simulink model "CHB_Rectifier"  (R2023b)
settings: Solver=FixedStepAuto  StartTime=0.0  StopTime=0.5  RelTol=1e-3
libraries: spsSeriesRLCBranchLib x4, spsVoltageMeasurementLib x4, spsMeanLib x3, spsParallelRLCBranchLib x2, spsUniversalBridgeLib x2, spsACVoltageSourceLib x1, spsCurrentMeasurementLib x1, slpidlib x1, powerlib_extras x1, spsRMSLib x1, spsTHDLib x1, spspowerguiLib x1
settings Model: SimulationMode=accelerator  Creator=abc6820292  LastModifiedBy=Epiphanye
settings SolverCC: ZeroCrossControl=EnableAll  ZeroCrossAlgorithm=Adaptive
settings DataIOCC: ReturnWorkspaceOutputs=off  Refine=10
settings DebuggingCC: IgnoredZcDiagnostic=none  UnconnectedInputMsg=warning  UnconnectedOutputMsg=warning  UnconnectedLineMsg=warning
settings ModelReferenceCC: EnableRefExpFcnMdlSchedulingChecks=on
settings RTWCC: DLArmComputeVersion=19.05

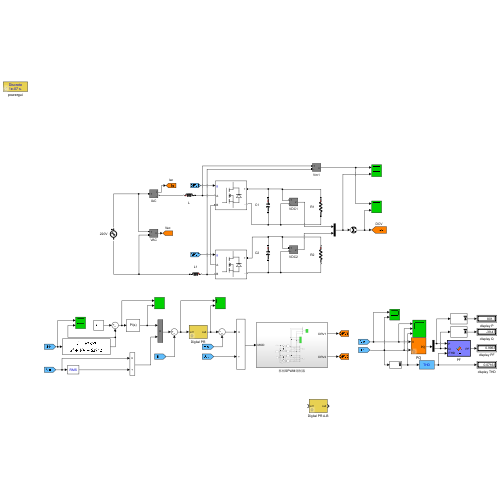
[thumbnail: Simulink's stored preview of the top-level diagram]
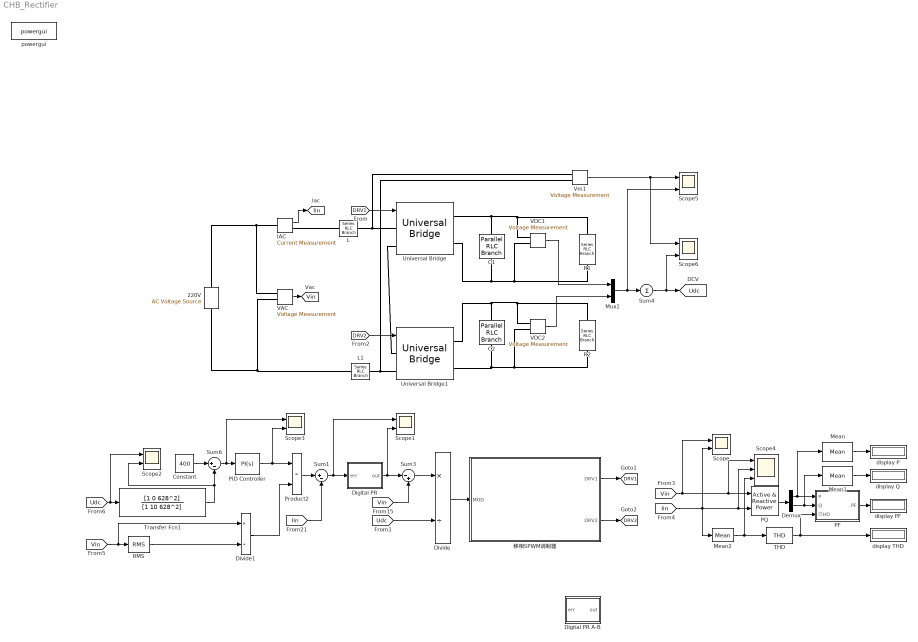
== system CHB_Rectifier ==
  220V : spsACVoltageSourceLib/AC Voltage Source  Amplitude=220*1.414  Phase=0  Frequency=50  SampleTime=0  Measurements=None  BusType=swing  Pref=10e3  Qref=0  Qmin=-inf  Qmax=+inf
  C1 : spsParallelRLCBranchLib/Parallel RLC Branch  LConnTagsString=a  RConnTagsString=__new0  BranchType=C  Resistance=1e3  Inductance=1e-3  SetiL0=off  InitialCurrent=0  Capacitance=1e-3  Setx0=on  InitialVoltage=80  Measurements=None
  C2 : spsParallelRLCBranchLib/Parallel RLC Branch  LConnTagsString=a  RConnTagsString=__new0  BranchType=C  Resistance=1e3  Inductance=1e-3  SetiL0=off  InitialCurrent=0  Capacitance=1e-3  Setx0=on  InitialVoltage=80  Measurements=None
  Constant : Constant  Value=400
  Demux : Demux  Outputs=2
  Digital PR : Subsystem  mask{Kp=8, Kr=100, Wc=5, Ts=1/40000, Upper=400, Lower=-400}
      mask DialogControl ParameterGroupVar Prompt: 参数
  Digital PR A-B : Subsystem  mask{Kp=6, Kr=400, Wc=5, Ts=1/20000, Upper=500, Lower=-500}
      mask DialogControl ParameterGroupVar Prompt: 参数
  Divide : Product  Inputs=*/
  Divide1 : Product  Inputs=*/
  IAC : spsCurrentMeasurementLib/Current Measurement  PhasorSimulation=off  OutputType=Complex  PSBequivalent=0
  L : spsSeriesRLCBranchLib/Series RLC Branch  LConnTagsString=__new0  RConnTagsString=__new0  BranchType=L  Resistance=25  Inductance=4e-4  SetiL0=off  InitialCurrent=0  Capacitance=2e-3  Setx0=on  InitialVoltage=350  Measurements=None
  L1 : spsSeriesRLCBranchLib/Series RLC Branch  LConnTagsString=__new0  RConnTagsString=__new0  BranchType=L  Resistance=25  Inductance=4e-4  SetiL0=off  InitialCurrent=0  Capacitance=2e-3  Setx0=on  InitialVoltage=350  Measurements=None
  Mean : spsMeanLib/Mean  Freq=50  Vinit=0  Ts=0
  Mean1 : spsMeanLib/Mean  Freq=50  Vinit=0  Ts=0
  Mean2 : spsMeanLib/Mean  Freq=20000  Vinit=0  Ts=0
  Mux1 : Mux  Inputs=2
  PF : MATLAB Function  TreatAsAtomicUnit=on
  PID Controller : slpidlib/PID Controller  Controller=PI  Form=Parallel  TimeDomain=Continuous-time  UseExternalTs=off  SampleTime=-1  IntegratorMethod=Forward Euler  FilterMethod=Forward Euler  ControllerParametersSource=internal  P=0.1  I=50  UseKiTs=off  D=0.005  N=100  UseFilter=on  TunerSelectOption=Transfer Function Based (PID Tuner App)  InitialConditionSource=internal  InitialConditionForIntegrator=0  InitialConditionForFilter=0  DifferentiatorICPrevScaledInput=0  ExternalReset=none  TrackingMode=off  Kt=1  LimitOutput=off  SatLimitsSource=internal  UpperSaturationLimit=40  LowerSaturationLimit=-20  LinearizeAsGain=on  AntiWindupMode=clamping  Kb=1  LimitIntegrator=off  UpperIntegratorSaturationLimit=inf  LowerIntegratorSaturationLimit=-inf  POutMin=[]  POutMax=[]  IOutMin=[]  IOutMax=[]  DOutMin=[]  DOutMax=[]  NOutMin=[]  NOutMax=[]  SumOutMin=[]  SumOutMax=[]  SaturationOutMin=[]  SaturationOutMax=[]  PParamMin=[]  PParamMax=[]  IParamMin=[]  IParamMax=[]  DParamMin=[]  DParamMax=[]  NParamMin=[]  NParamMax=[]  KbParamMin=[]  KbParamMax=[]  KtParamMin=[]  KtParamMax=[]  KbOutMin=[]  KbOutMax=[]  KtOutMin=[]  KtOutMax=[]  IntegratorOutMin=[]  IntegratorOutMax=[]  FilterOutMin=[]  FilterOutMax=[]  SumI1OutMin=[]  SumI1OutMax=[]  SumI2OutMin=[]  SumI2OutMax=[]  SumI3OutMin=[]  SumI3OutMax=[]  SumI4OutMin=[]  SumI4OutMax=[]  SumDOutMin=[]  SumDOutMax=[]  DifferentiatorOutMin=[]  DifferentiatorOutMax=[]  FilterDiffOutCoefMin=[]  FilterDiffOutCoefMax=[]  ReciprocalOutMin=[]  ReciprocalOutMax=[]  SumDenOutMin=[]  SumDenOutMax=[]  SumNumOutMin=[]  SumNumOutMax=[]  DivideOutMin=[]  DivideOutMax=[]  UdiffTsProdOutMin=[]  UdiffTsProdOutMax=[]  NTsProdOutMin=[]  NTsProdOutMax=[]  UintegralTsProdOutMin=[]  UintegralTsProdOutMax=[]  UngainTsProdOutMin=[]  UngainTsProdOutMax=[]  ClampingZeroOutDataTypeStr=Inherit: Inherit via back propagation  ClampingZeroOutMin=[]  ClampingZeroOutMax=[]  FilterDenConstantOutDataTypeStr=Inherit: Inherit via back propagation  FilterDenConstantOutMin=[]  FilterDenConstantOutMax=[]  PCopyOutDataTypeStr=Inherit: Inherit via back propagation  PCopyOutMin=[]  PCopyOutMax=[]  NCopyOutDataTypeStr=Inherit: Inherit via back propagation  NCopyOutMin=[]  NCopyOutMax=[]  IntegratorContinuousStateAttributes=''  IntegratorStateMustResolveToSignalObject=off  IntegratorRTWStateStorageClass=Auto  FilterContinuousStateAttributes=''  FilterStateMustResolveToSignalObject=off  FilterRTWStateStorageClass=Auto  ParallelPVariant=InternalParameters  IdealPVariant=Disabled  IVariant=InternalParameters  DVariant=Disabled  IntegratorVariant=Continuous  SatVariant=Disabled  AWVariant=Passthrough  PCopyVariant=Disabled  TRVariant=Disabled  FdbkBlocksVariant=Forward  IdealPFdbkVariant=Disabled  SatFdbkVariant=Disabled  DerivativeFilterVariant=Disabled  NVariant=Disabled  NCopyVariant=Disabled_SignalSpec  FilterICVariant=Disabled  IntegratorICVariant=InternalICs  ExternalResetVariant=Disabled  TRSumVariant=Passthrough  SumFdbkVariant=Disabled  SumVariant=Sum_PI  TsampFilterVariant=InternalTs  TsampNgainVariant=Passthrough  TsampIntegralVariant=Disabled_SignalSpec  ExternalSaturationOutDataTypeStr=Inherit: Same as second input
  PQ : powerlib_extras/Measurements/Active & Reactive Power  f1=50
  Product2 : Product  RndMeth=Zero
  R1 : spsSeriesRLCBranchLib/Series RLC Branch  LConnTagsString=__new0  RConnTagsString=__new0  BranchType=R  Resistance=100  Inductance=0.1  SetiL0=off  InitialCurrent=0  Capacitance=2e-3  Setx0=on  InitialVoltage=350  Measurements=None
  R2 : spsSeriesRLCBranchLib/Series RLC Branch  LConnTagsString=__new0  RConnTagsString=__new0  BranchType=R  Resistance=100  Inductance=0.1  SetiL0=off  InitialCurrent=0  Capacitance=2e-3  Setx0=on  InitialVoltage=350  Measurements=None
  RMS : spsRMSLib/RMS  TrueRMS=on  Freq=60  RMSInit=120  Ts=0
  Scope{,1..3,5..6} (6 alike) : Scope  NumInputPorts=2
  Scope4 : Scope  NumInputPorts=3
  Sum1 : Sum  Inputs=|+-
  Sum3 : Sum  Inputs=|-+
  Sum4 : Sum  Inputs=+
  Sum6 : Sum  Inputs=|+-
  THD : spsTHDLib/THD  Freq=50  Ts=0
  Transfer Fcn1 : TransferFcn  Numerator=[1 0 628^2]  Denominator=[1 10 628^2]
  Universal Bridge : spsUniversalBridgeLib/Universal Bridge  Arms=2  SnubberResistance=1e5  SnubberCapacitance=inf  Device=MOSFET / Diodes  Ron=1e-3  Lon=0  ForwardVoltages="[  0  0  ]"  ForwardVoltage=0  GTOparameters=[ 10e-6 , 20e-6 ]  IGBTparameters=[ 1e-6 , 2e-6 ]  Measurements=None  Measurements_2=None  converterType=Rectifier
  Universal Bridge1 : spsUniversalBridgeLib/Universal Bridge  Arms=2  SnubberResistance=1e5  SnubberCapacitance=inf  Device=MOSFET / Diodes  Ron=1e-3  Lon=0  ForwardVoltages="[  0  0  ]"  ForwardVoltage=0  GTOparameters=[ 10e-6 , 20e-6 ]  IGBTparameters=[ 1e-6 , 2e-6 ]  Measurements=None  Measurements_2=None  converterType=Rectifier
  VAC : spsVoltageMeasurementLib/Voltage Measurement  PhasorSimulation=off  OutputType=Complex  PSBequivalent=0
  VDC1 : spsVoltageMeasurementLib/Voltage Measurement  PhasorSimulation=off  OutputType=Complex  PSBequivalent=0
  VDC2 : spsVoltageMeasurementLib/Voltage Measurement  PhasorSimulation=off  OutputType=Complex  PSBequivalent=0
  Vm1 : spsVoltageMeasurementLib/Voltage Measurement  PhasorSimulation=off  OutputType=Complex  PSBequivalent=0
  display P : Display
  display PF : Display
  display Q : Display
  display THD : Display
  powergui : spspowerguiLib/powergui  SimulationMode=Discrete  SampleTime=1e-7  frequency=60  Iterations=50  frequencyindice=0  Pbase=100e6  ErrMax=1e-4  UnitsV=kV  UnitsW=MW  buscounter=0  FunctionMessages=off  echomessages=off  EnableUseOfTLC=off  CurrentSourceSwitches=off  DisableSnubberDevices=off  DisableRonSwitches=off  DisableVfSwitches=off  DisplayEquations=off  AutomaticDiscreteSolvers=off  SolverType=Tustin/Backward Euler (TBE)  Interpol=off  ExternalGateDelay=off  methode=off  Ts=0  x0status=blocks  SPID=off  SwTol=0  HookPort=off  NonlinearTolerance=1e-4  nMaxIteration=100  ContinueOnMaxIteration=off  RestoreLinks=warning  ResistiveCurrentMeasurement=off  Frange=[0:2:500]  Ylog=off  Xlog=on  ShowGrid=off  save=off  variable=ZData  structure=QQQQQ  ZoomFFT=off  StartTime=0.5  cycles=15  DisplayStyle=1  fundamental=50  FreqAxis=off  MaxFrequency=1000  frequencyindicesteady=1  RmsSteady=1  display=off
  移相SPWM调制器 : Subsystem
  tag scope: DRV1=global, DRV2=global, Iin=global, Udc=global, Vin=global
  wires:
  VAC/1 -> [Vin]
  [Vin] -> Scope/1, Scope4/1, PQ/1
  PQ/1 -> Demux/1
  Demux/1 -> Mean/1, PF/1(P)
  Demux/2 -> Mean1/1, PF/2(Q)
  THD/1 -> display THD/1, PF/3(iTHD)
  PF/1(PF) -> display PF/1
  Mean/1 -> display P/1
  Mean1/1 -> display Q/1
  [DRV1] -> Universal Bridge/1
  移相SPWM调制器/1(DRV1) -> [DRV1]
  IAC/1 -> [Iin]
  [Iin] -> Scope/2, Mean2/1, Scope4/2, PQ/2
  Mean2/1 -> Scope4/3, THD/1
  Sum1/1 -> Digital PR/1(err), Scope1/1
  Product2/1 -> Sum1/1
  PID Controller/1 -> Scope3/2, Product2/1
  Sum3/1 -> Divide/1
  Sum6/1 -> Scope3/1, PID Controller/1
  Constant/1 -> Sum6/1
  Vm1/1 -> Scope6/1, Scope5/1
  [DRV2] -> Universal Bridge1/1
  VDC1/1 -> Mux1/1
  VDC2/1 -> Mux1/2
  Mux1/1 -> Scope5/2, Sum4/1
  Sum4/1 -> Scope6/2, [Udc]
  Digital PR/1(out) -> Scope1/2, Sum3/1
  [Udc] -> Divide/2
  移相SPWM调制器/2(DRV2) -> [DRV2]
  Divide/1 -> 移相SPWM调制器/1(MOD)
  [Vin] -> Sum3/2
  [Vin] -> Divide1/1, RMS/1
  RMS/1 -> Divide1/2
  Divide1/1 -> Product2/2
  [Iin] -> Sum1/2
  [Udc] -> Scope2/1, Transfer Fcn1/1
  Transfer Fcn1/1 -> Scope2/2, Sum6/2
  connections:
  Universal Bridge/RConn2 -- VDC1/LConn2 -- R1/RConn1 -- C1/RConn1
  IAC/LConn1 -- VAC/LConn1 -- 220V/RConn1
  C1/LConn1 -- R1/LConn1 -- VDC1/LConn1 -- Universal Bridge/RConn1
  L/RConn1 -- Universal Bridge/LConn1 -- Vm1/LConn1
  L/LConn1 -- IAC/RConn1
  L1/RConn1 -- 220V/LConn1 -- VAC/LConn2
  Universal Bridge/LConn2 -- Universal Bridge1/LConn1
  VDC2/LConn2 -- R2/RConn1 -- Universal Bridge1/RConn2 -- C2/RConn1
  C2/LConn1 -- Universal Bridge1/RConn1 -- VDC2/LConn1 -- R2/LConn1
  Vm1/LConn2 -- L1/LConn1 -- Universal Bridge1/LConn2

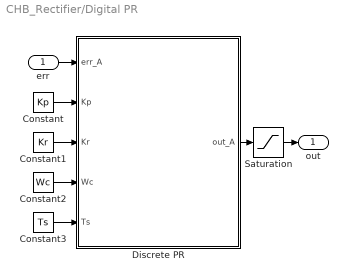
== system CHB_Rectifier/Digital PR ==
  err : Inport
  Constant : Constant  Value=Kp
  Constant1 : Constant  Value=Kr
  Constant2 : Constant  Value=Wc
  Constant3 : Constant  Value=Ts
  Discrete PR : MATLAB Function  TreatAsAtomicUnit=on
  Saturation : Saturate  UpperLimit=Upper  LowerLimit=Lower
  out : Outport
  wires:
  Constant1/1 -> Discrete PR/3(Kr)
  Constant3/1 -> Discrete PR/5(Ts)
  Constant/1 -> Discrete PR/2(Kp)
  Constant2/1 -> Discrete PR/4(Wc)
  Discrete PR/1(out_A) -> Saturation/1
  Saturation/1 -> out/1
  err/1 -> Discrete PR/1(err_A)

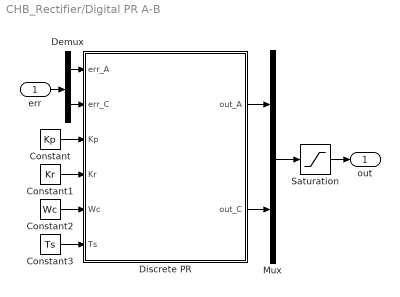
== system CHB_Rectifier/Digital PR A-B ==
  err : Inport
  Constant : Constant  Value=Kp
  Constant1 : Constant  Value=Kr
  Constant2 : Constant  Value=Wc
  Constant3 : Constant  Value=Ts
  Demux : Demux  Outputs=2
  Discrete PR : MATLAB Function  TreatAsAtomicUnit=on
  Mux : Mux  Inputs=2
  Saturation : Saturate  UpperLimit=Upper  LowerLimit=Lower
  out : Outport
  wires:
  Constant1/1 -> Discrete PR/4(Kr)
  Constant3/1 -> Discrete PR/6(Ts)
  Constant/1 -> Discrete PR/3(Kp)
  Constant2/1 -> Discrete PR/5(Wc)
  Demux/1 -> Discrete PR/1(err_A)
  err/1 -> Demux/1
  Demux/2 -> Discrete PR/2(err_C)
  Discrete PR/1(out_A) -> Mux/1
  Discrete PR/2(out_C) -> Mux/2
  Mux/1 -> Saturation/1
  Saturation/1 -> out/1

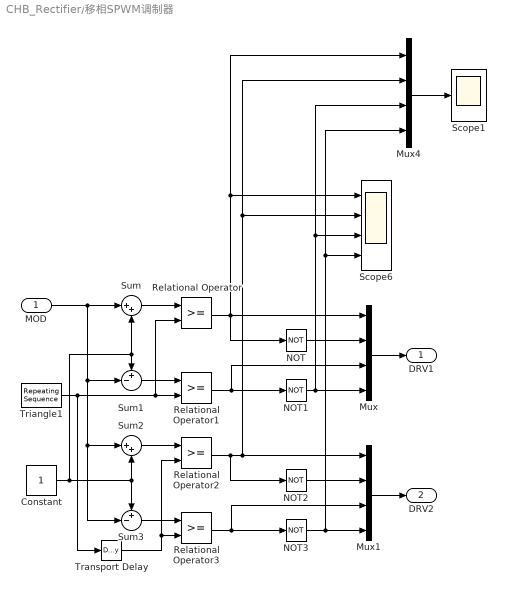
== system CHB_Rectifier/移相SPWM调制器 ==
  MOD : Inport
  Constant : Constant
  Mux : Mux
  Mux1 : Mux
  Mux4 : Mux
  NOT{,1..3} (4 alike) : Logic  Operator=NOT  IconShape=distinctive  AllPortsSameDT=off  OutDataTypeStr=boolean
  Relational Operator{,1..3} (4 alike) : RelationalOperator  OutDataTypeStr=boolean  InputSameDT=off
  Scope1 : Scope
  Scope6 : Scope  NumInputPorts=4
  Sum : Sum  Inputs=|++
  Sum1 : Sum  Inputs=+-|
  Sum2 : Sum  Inputs=|++
  Sum3 : Sum  Inputs=+-|
  Transport Delay : TransportDelay  DelayTime=1/20000/4
  Triangle1 : simulink/Sources/Repeating Sequence  rep_seq_t=[0 1/20000/2 1/20000]  rep_seq_y=[0 2 0]
  DRV1 : Outport
  DRV2 : Outport  Port=2
  wires:
  Triangle1/1 -> Transport Delay/1, Relational Operator1/2, Relational Operator/2
  Mux/1 -> DRV1/1
  NOT/1 -> Mux/2
  Relational Operator/1 -> Mux4/1, Scope6/1, Mux/1, NOT/1
  MOD/1 -> Sum3/2, Sum2/1, Sum1/2, Sum/1
  Sum/1 -> Relational Operator/1
  Sum1/1 -> Relational Operator1/1
  Relational Operator1/1 -> Mux/3, NOT1/1
  Constant/1 -> Sum3/1, Sum2/2, Sum/2, Sum1/1
  NOT1/1 -> Mux4/3, Scope6/3, Mux/4
  Relational Operator3/1 -> Mux1/3, NOT3/1
  Relational Operator2/1 -> Mux1/1, Mux4/2, Scope6/2, NOT2/1
  NOT2/1 -> Mux1/2
  NOT3/1 -> Mux4/4, Scope6/4, Mux1/4
  Sum3/1 -> Relational Operator3/1
  Sum2/1 -> Relational Operator2/1
  Transport Delay/1 -> Relational Operator3/2, Relational Operator2/2
  Mux1/1 -> DRV2/1
  Mux4/1 -> Scope1/1

== matlab function CHB_Rectifier/Digital PR/Discrete PR ==
  settings: updateMethod=DISCRETE  sampleTime=Ts
  data: err_A input; out_A output; Kp input; Kr input; Wc input; Ts input
function out_A  = fcn(err_A, Kp, Kr, Wc, Ts)

W0 = 50*2*pi;


persistent err_A1;
persistent err_A2;
persistent out_A1;
persistent out_A2;


%%对三相静态变量初始化
if isempty(err_A1)
    err_A1 = 0;
end
if isempty(err_A2)
    err_A2 = 0;
end
if isempty(out_A1)
    out_A1 = 0;
end
if isempty(out_A2)
    out_A2 = 0;
end


%%Discrete
t1 = Wc * Ts;
t2 = W0^2 * Ts^2;
t3 = t2 + 4*t1 + 4;

b0 = (Kp*t2 + 4*(Kp+Kr)*t1 + 4*Kp) / t3;
b1 = (2*Kp*t2 - 8*Kp) / t3;
b2 = (Kp*t2 + 4*Kp - 4*(Kp+Kr)*t1) / t3;
a1 = (2*t2 - 8) / t3;
a2 = (t2 - 4*t1 + 4) / t3;
%%限制输出
if b0>3000
    b0=0;
end
if b0<-3000
    b0=0;
end

%%计算输出量
out_A = b0*err_A + b1*err_A1 + b2*err_A2 - a1*out_A1 - a2*out_A2;
out_A2 = out_A1;
out_A1 = out_A;
err_A2 = err_A1;
err_A1 = err_A;

== matlab function CHB_Rectifier/PF ==
  data: P input; PF output; Q input; iTHD input
function PF = fcn(P,Q,iTHD)
% This block supports an embeddable subset of the MATLAB language.
% See the help menu for details. 
PF=(P/sqrt(P*P+Q*Q))/(sqrt(1+iTHD*iTHD));

== matlab function CHB_Rectifier/Digital PR A-B/Discrete PR ==
  settings: updateMethod=DISCRETE  sampleTime=Ts
  data: err_A input; err_C input; out_A output; Kp input; Kr input; Wc input; Ts input; out_C output
function [out_A, out_C] = fcn(err_A, err_C, Kp, Kr, Wc, Ts)

W0 = 50*2*pi;

%%定义三相静态变量
persistent err_A1;
persistent err_A2;
persistent out_A1;
persistent out_A2;

persistent err_C1;
persistent err_C2;
persistent out_C1;
persistent out_C2;

%%对三相静态变量初始化
if isempty(err_A1)
    err_A1 = 0;
end
if isempty(err_A2)
    err_A2 = 0;
end
if isempty(out_A1)
    out_A1 = 0;
end
if isempty(out_A2)
    out_A2 = 0;
end


if isempty(err_C1)
    err_C1 = 0;
end
if isempty(err_C2)
    err_C2 = 0;
end
if isempty(out_C1)
    out_C1 = 0;
end
if isempty(out_C2)
    out_C2 = 0;
end

%%Discrete
t1 = Wc * Ts;
t2 = W0^2 * Ts^2;
t3 = t2 + 4*t1 + 4;

b0 = (Kp*t2 + 4*(Kp+Kr)*t1 + 4*Kp) / t3;
b1 = (2*Kp*t2 - 8*Kp) / t3;
b2 = (Kp*t2 + 4*Kp - 4*(Kp+Kr)*t1) / t3;
a1 = (2*t2 - 8) / t3;
a2 = (t2 - 4*t1 + 4) / t3;

%%计算三相输出量
out_A = b0*err_A + b1*err_A1 + b2*err_A2 - a1*out_A1 - a2*out_A2;
out_A2 = out_A1;
out_A1 = out_A;
err_A2 = err_A1;
err_A1 = err_A;


out_C = b0*err_C + b1*err_C1 + b2*err_C2 - a1*out_C1 - a2*out_C2;
out_C2 = out_C1;
out_C1 = out_C;
err_C2 = err_C1;
err_C1 = err_C;
